simulink library "Load_Lib"  (R2025a)
settings: Solver=ode45  StartTime=0.0  StopTime=10.0  RelTol=1e-3  EnableMultiTasking=on
undefined symbols (not defined in the file or in its folder): Local, Scissor_Lift_Param, X, Y, Z
libraries: sm_lib x41, Scissor_Parts_Lib x24, fl_lib x6
(part 1 of 2)
Description:
  | Copyright 2015-2025 The MathWorks, Inc.
settings Model: Creator=smiller  LastModifiedBy=smiller
settings SolverCC: AlgebraicLoopSolver=TrustRegion
settings DataIOCC: LimitDataPoints=on  SaveFormat=Array  ReturnWorkspaceOutputs=off
settings OptimizationCC: ReuseModelBlockBuffer=off  ExpressionDepthLimit=2147483647.0  LifeSpan=inf
settings DebuggingCC: UnderspecifiedInitializationDetection=Classic  MergeDetectMultiDrivingBlocksExec=none  SolverPrmCheckMsg=warning  UnconnectedInputMsg=warning  UnconnectedOutputMsg=warning  UnconnectedLineMsg=warning  AllowSymbolicDim=off  StateNameClashWarn=warning  PregeneratedLibrarySubsystemCodeDiagnostic=none  SFUnexpectedBacktrackingDiag=warning  SFNoUnconditionalDefaultTransitionDiag=warning  SFExecutionAtInitializationDiag=none  ArithmeticOperatorsInVariantConditions=warning
settings HardwareCC: ProdBitPerPointer=32.0  ProdBitPerSizeT=32.0  ProdBitPerPtrDiffT=32.0  ProdLargestAtomicFloat=None  ProdIntDivRoundTo=Undefined  ProdEndianess=Unspecified  ProdWordSize=32.0  ProdHWDeviceType=32-bit Generic
settings ModelReferenceCC: EnableRefExpFcnMdlSchedulingChecks=on  PropagateSignalLabelsOutOfModel=off
settings SFSimCC: SimUseLocalCustomCode=off  CustomCodeUndefinedFunction=UseInterfaceOnly
settings RTWCC: RTWUseLocalCustomCode=off  GPUComputeCapability=3.5  DLArmComputeVersion=19.05
settings CodeAppCC: StateflowObjectComments=on
settings GRTTargetCC: TargetLangStandard=C89/C90 (ANSI)
settings ConfigComp: CovMetricSettings=dw  CovSaveCumulativeToWorkspaceVar=on  CovSaveSingleToWorkspaceVar=on  CovExternalEMLEnable=off  CovSFcnEnable=off

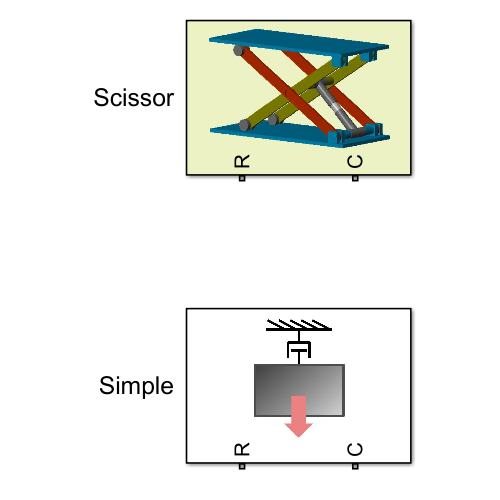
[thumbnail: Simulink's stored preview of the top-level diagram]
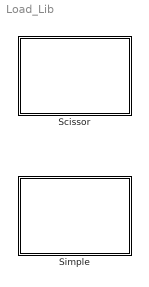
== system Load_Lib ==
  Scissor : Subsystem
      mask Display: image('Load_Scissor_IMAGE.JPG');
  Simple : Subsystem
      mask Display: image('Load_Simple_IMAGE.JPG');

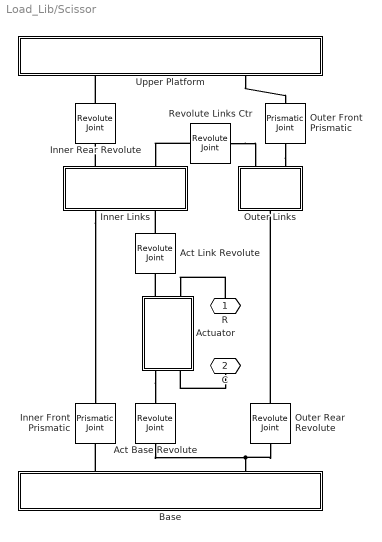
== system Load_Lib/Scissor ==
  Act Base Revolute : sm_lib/Joints/Revolute Joint  JointMode=Normal  CompositeWrenchDir=FollowerOnBase  CompositeWrenchFrame=BaseFrame  SenseConstraintForce=off  SenseConstraintTorque=off  SenseTotalForce=off  SenseTotalTorque=off  PositionTargetSpecify=off  PositionTargetPriority=High  PositionTargetValue=0  PositionTargetValueUnits=deg  VelocityTargetSpecify=off  VelocityTargetPriority=High  VelocityTargetValue=0  VelocityTargetValueUnits=deg/s  EquilibriumPosition=0  EquilibriumPositionUnits=deg  SpringStiffness=0  SpringStiffnessUnits=N*m/deg  DampingCoefficient=0  DampingCoefficientUnits=N*m/(deg/s)  LowerLimitSpecify=off  LowerLimitBound=-90  LowerLimitBoundUnits=deg  LowerLimitStiffness=1e4  LowerLimitStiffnessUnits=N*m/deg  LowerLimitDamping=10  LowerLimitDampingUnits=N*m/(deg/s)  LowerLimitTransitionRegionWidth=0.1  LowerLimitTransitionRegionWidthUnits=deg  UpperLimitSpecify=off  UpperLimitBound=90  UpperLimitBoundUnits=deg  UpperLimitStiffness=1e4  UpperLimitStiffnessUnits=N*m/deg  UpperLimitDamping=10  UpperLimitDampingUnits=N*m/(deg/s)  UpperLimitTransitionRegionWidth=0.1  UpperLimitTransitionRegionWidthUnits=deg  TorqueActuationMode=NoTorque  MotionActuationMode=ComputedMotion  SensePosition=off  SenseVelocity=off  SenseAcceleration=off  SenseTorqueForce=off  SenseLowerLimitTorqueForce=off  SenseUpperLimitTorqueForce=off
  Act Link Revolute : sm_lib/Joints/Revolute Joint  JointMode=Normal  CompositeWrenchDir=FollowerOnBase  CompositeWrenchFrame=BaseFrame  SenseConstraintForce=off  SenseConstraintTorque=off  SenseTotalForce=off  SenseTotalTorque=off  PositionTargetSpecify=off  PositionTargetPriority=High  PositionTargetValue=0  PositionTargetValueUnits=deg  VelocityTargetSpecify=off  VelocityTargetPriority=High  VelocityTargetValue=0  VelocityTargetValueUnits=deg/s  EquilibriumPosition=0  EquilibriumPositionUnits=deg  SpringStiffness=0  SpringStiffnessUnits=N*m/deg  DampingCoefficient=0  DampingCoefficientUnits=N*m/(deg/s)  LowerLimitSpecify=off  LowerLimitBound=-90  LowerLimitBoundUnits=deg  LowerLimitStiffness=1e4  LowerLimitStiffnessUnits=N*m/deg  LowerLimitDamping=10  LowerLimitDampingUnits=N*m/(deg/s)  LowerLimitTransitionRegionWidth=0.1  LowerLimitTransitionRegionWidthUnits=deg  UpperLimitSpecify=off  UpperLimitBound=90  UpperLimitBoundUnits=deg  UpperLimitStiffness=1e4  UpperLimitStiffnessUnits=N*m/deg  UpperLimitDamping=10  UpperLimitDampingUnits=N*m/(deg/s)  UpperLimitTransitionRegionWidth=0.1  UpperLimitTransitionRegionWidthUnits=deg  TorqueActuationMode=NoTorque  MotionActuationMode=ComputedMotion  SensePosition=off  SenseVelocity=off  SenseAcceleration=off  SenseTorqueForce=off  SenseLowerLimitTorqueForce=off  SenseUpperLimitTorqueForce=off
  Actuator : Subsystem
  Base : Subsystem
  Inner Links : Subsystem
  "Inner Front Prismatic " : sm_lib/Joints/Prismatic Joint  JointMode=Normal  CompositeWrenchDir=FollowerOnBase  CompositeWrenchFrame=BaseFrame  SenseConstraintForce=off  SenseConstraintTorque=off  SenseTotalForce=off  SenseTotalTorque=off  PositionTargetSpecify=off  PositionTargetPriority=High  PositionTargetValue=0  PositionTargetValueUnits=m  VelocityTargetSpecify=off  VelocityTargetPriority=High  VelocityTargetValue=0  VelocityTargetValueUnits=m/s  EquilibriumPosition=0  EquilibriumPositionUnits=m  SpringStiffness=0  SpringStiffnessUnits=N/m  DampingCoefficient=0  DampingCoefficientUnits=N/(m/s)  LowerLimitSpecify=off  LowerLimitBound=-1  LowerLimitBoundUnits=m  LowerLimitStiffness=1e6  LowerLimitStiffnessUnits=N/m  LowerLimitDamping=1e3  LowerLimitDampingUnits=N/(m/s)  LowerLimitTransitionRegionWidth=1e-4  LowerLimitTransitionRegionWidthUnits=m  UpperLimitSpecify=off  UpperLimitBound=1  UpperLimitBoundUnits=m  UpperLimitStiffness=1e6  UpperLimitStiffnessUnits=N/m  UpperLimitDamping=1e3  UpperLimitDampingUnits=N/(m/s)  UpperLimitTransitionRegionWidth=1e-4  UpperLimitTransitionRegionWidthUnits=m  TorqueActuationMode=NoTorque  MotionActuationMode=ComputedMotion  SensePosition=off  SenseVelocity=off  SenseAcceleration=off  SenseTorqueForce=off  SenseLowerLimitTorqueForce=off  SenseUpperLimitTorqueForce=off
  Inner Rear Revolute : sm_lib/Joints/Revolute Joint  JointMode=Normal  CompositeWrenchDir=FollowerOnBase  CompositeWrenchFrame=BaseFrame  SenseConstraintForce=off  SenseConstraintTorque=off  SenseTotalForce=off  SenseTotalTorque=off  PositionTargetSpecify=off  PositionTargetPriority=Low  PositionTargetValue=15  PositionTargetValueUnits=deg  VelocityTargetSpecify=off  VelocityTargetPriority=High  VelocityTargetValue=0  VelocityTargetValueUnits=deg/s  EquilibriumPosition=0  EquilibriumPositionUnits=deg  SpringStiffness=0  SpringStiffnessUnits=N*m/deg  DampingCoefficient=0  DampingCoefficientUnits=N*m/(deg/s)  LowerLimitSpecify=off  LowerLimitBound=-90  LowerLimitBoundUnits=deg  LowerLimitStiffness=1e4  LowerLimitStiffnessUnits=N*m/deg  LowerLimitDamping=10  LowerLimitDampingUnits=N*m/(deg/s)  LowerLimitTransitionRegionWidth=0.1  LowerLimitTransitionRegionWidthUnits=deg  UpperLimitSpecify=off  UpperLimitBound=90  UpperLimitBoundUnits=deg  UpperLimitStiffness=1e4  UpperLimitStiffnessUnits=N*m/deg  UpperLimitDamping=10  UpperLimitDampingUnits=N*m/(deg/s)  UpperLimitTransitionRegionWidth=0.1  UpperLimitTransitionRegionWidthUnits=deg  TorqueActuationMode=NoTorque  MotionActuationMode=ComputedMotion  SensePosition=off  SenseVelocity=off  SenseAcceleration=off  SenseTorqueForce=off  SenseLowerLimitTorqueForce=off  SenseUpperLimitTorqueForce=off
  Outer Links : Subsystem
  "Outer Front Prismatic " : sm_lib/Joints/Prismatic Joint  JointMode=Normal  CompositeWrenchDir=FollowerOnBase  CompositeWrenchFrame=BaseFrame  SenseConstraintForce=off  SenseConstraintTorque=off  SenseTotalForce=off  SenseTotalTorque=off  PositionTargetSpecify=off  PositionTargetPriority=High  PositionTargetValue=0  PositionTargetValueUnits=m  VelocityTargetSpecify=off  VelocityTargetPriority=High  VelocityTargetValue=0  VelocityTargetValueUnits=m/s  EquilibriumPosition=0  EquilibriumPositionUnits=m  SpringStiffness=0  SpringStiffnessUnits=N/m  DampingCoefficient=0  DampingCoefficientUnits=N/(m/s)  LowerLimitSpecify=off  LowerLimitBound=-1  LowerLimitBoundUnits=m  LowerLimitStiffness=1e6  LowerLimitStiffnessUnits=N/m  LowerLimitDamping=1e3  LowerLimitDampingUnits=N/(m/s)  LowerLimitTransitionRegionWidth=1e-4  LowerLimitTransitionRegionWidthUnits=m  UpperLimitSpecify=off  UpperLimitBound=1  UpperLimitBoundUnits=m  UpperLimitStiffness=1e6  UpperLimitStiffnessUnits=N/m  UpperLimitDamping=1e3  UpperLimitDampingUnits=N/(m/s)  UpperLimitTransitionRegionWidth=1e-4  UpperLimitTransitionRegionWidthUnits=m  TorqueActuationMode=NoTorque  MotionActuationMode=ComputedMotion  SensePosition=off  SenseVelocity=off  SenseAcceleration=off  SenseTorqueForce=off  SenseLowerLimitTorqueForce=off  SenseUpperLimitTorqueForce=off
  Outer Rear Revolute : sm_lib/Joints/Revolute Joint  JointMode=Normal  CompositeWrenchDir=FollowerOnBase  CompositeWrenchFrame=BaseFrame  SenseConstraintForce=off  SenseConstraintTorque=off  SenseTotalForce=off  SenseTotalTorque=off  PositionTargetSpecify=off  PositionTargetPriority=Low  PositionTargetValue=-15  PositionTargetValueUnits=deg  VelocityTargetSpecify=off  VelocityTargetPriority=High  VelocityTargetValue=0  VelocityTargetValueUnits=deg/s  EquilibriumPosition=0  EquilibriumPositionUnits=deg  SpringStiffness=0  SpringStiffnessUnits=N*m/deg  DampingCoefficient=0  DampingCoefficientUnits=N*m/(deg/s)  LowerLimitSpecify=off  LowerLimitBound=-90  LowerLimitBoundUnits=deg  LowerLimitStiffness=1e4  LowerLimitStiffnessUnits=N*m/deg  LowerLimitDamping=10  LowerLimitDampingUnits=N*m/(deg/s)  LowerLimitTransitionRegionWidth=0.1  LowerLimitTransitionRegionWidthUnits=deg  UpperLimitSpecify=off  UpperLimitBound=90  UpperLimitBoundUnits=deg  UpperLimitStiffness=1e4  UpperLimitStiffnessUnits=N*m/deg  UpperLimitDamping=10  UpperLimitDampingUnits=N*m/(deg/s)  UpperLimitTransitionRegionWidth=0.1  UpperLimitTransitionRegionWidthUnits=deg  TorqueActuationMode=NoTorque  MotionActuationMode=ComputedMotion  SensePosition=off  SenseVelocity=off  SenseAcceleration=off  SenseTorqueForce=off  SenseLowerLimitTorqueForce=off  SenseUpperLimitTorqueForce=off
  Revolute Links Ctr : sm_lib/Joints/Revolute Joint  JointMode=Normal  CompositeWrenchDir=FollowerOnBase  CompositeWrenchFrame=BaseFrame  SenseConstraintForce=off  SenseConstraintTorque=off  SenseTotalForce=off  SenseTotalTorque=off  PositionTargetSpecify=on  PositionTargetPriority=Low  PositionTargetValue=-2*Scissor_Lift_Param.Initial_Angle  PositionTargetValueUnits=deg  VelocityTargetSpecify=off  VelocityTargetPriority=High  VelocityTargetValue=0  VelocityTargetValueUnits=deg/s  EquilibriumPosition=0  EquilibriumPositionUnits=deg  SpringStiffness=0  SpringStiffnessUnits=N*m/deg  DampingCoefficient=0  DampingCoefficientUnits=N*m/(deg/s)  LowerLimitSpecify=off  LowerLimitBound=-90  LowerLimitBoundUnits=deg  LowerLimitStiffness=1e4  LowerLimitStiffnessUnits=N*m/deg  LowerLimitDamping=10  LowerLimitDampingUnits=N*m/(deg/s)  LowerLimitTransitionRegionWidth=0.1  LowerLimitTransitionRegionWidthUnits=deg  UpperLimitSpecify=off  UpperLimitBound=90  UpperLimitBoundUnits=deg  UpperLimitStiffness=1e4  UpperLimitStiffnessUnits=N*m/deg  UpperLimitDamping=10  UpperLimitDampingUnits=N*m/(deg/s)  UpperLimitTransitionRegionWidth=0.1  UpperLimitTransitionRegionWidthUnits=deg  TorqueActuationMode=NoTorque  MotionActuationMode=ComputedMotion  SensePosition=off  SenseVelocity=off  SenseAcceleration=off  SenseTorqueForce=off  SenseLowerLimitTorqueForce=off  SenseUpperLimitTorqueForce=off
  Upper Platform : Subsystem
  R : PMIOPort  Side=Left
  C : PMIOPort  Port=2  Side=Left
  connections:
  R/RConn1 -- Actuator/RConn2
  C/RConn1 -- Actuator/LConn2
  Actuator/LConn1 -- Act Base Revolute/RConn1
  Act Link Revolute/LConn1 -- Inner Links/RConn2
  Actuator/RConn1 -- Act Link Revolute/RConn1
  Revolute Links Ctr/LConn1 -- Inner Links/LConn2
  Revolute Links Ctr/RConn1 -- Outer Links/RConn1
  Outer Rear Revolute/RConn1 -- Outer Links/LConn1
  Inner Links/LConn1 -- Inner Rear Revolute/RConn1
  Inner Rear Revolute/LConn1 -- Upper Platform/LConn1
  "Outer Front Prismatic "/LConn1 -- Outer Links/RConn2
  Upper Platform/LConn2 -- "Outer Front Prismatic "/RConn1
  Base/RConn1 -- "Inner Front Prismatic "/RConn1
  Inner Links/RConn1 -- "Inner Front Prismatic "/LConn1
  Outer Rear Revolute/LConn1 -- Base/RConn2 -- Act Base Revolute/LConn1

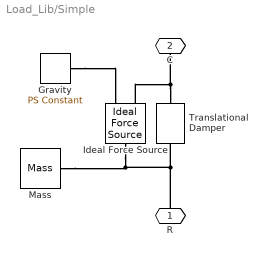
== system Load_Lib/Simple ==
  Gravity : fl_lib/Physical Signals/Sources/PS Constant  constant=9.81*Scissor_Lift_Param.Load.Mass N
  Ideal Force Source : fl_lib/Mechanical/Mechanical Sources/Ideal Force Source
  Mass : fl_lib/Mechanical/Translational Elements/Mass  mass=Scissor_Lift_Param.Load.Mass kg  num_ports=foundation.enum.numPorts2.one  v_specify=on  v_priority=High  v=0 m/s  v_nominal_specify=off  v_nominal_value=1  v_nominal_unit=m/s  f_specify=off  f_priority=High  f=0 N  f_nominal_specify=off  f_nominal_value=1  f_nominal_unit=N
  Translational Damper : fl_lib/Mechanical/Translational Elements/Translational Damper  D=Scissor_Lift_Param.Actuator.Damping N/(m/s)  v_specify=off  v_priority=High  v=0 m/s  v_nominal_specify=off  v_nominal_value=1  v_nominal_unit=m/s  f_specify=off  f_priority=High  f=0 N  f_nominal_specify=off  f_nominal_value=1  f_nominal_unit=N
  R : PMIOPort  Side=Left
  C : PMIOPort  Port=2  Side=Left
  connections:
  Translational Damper/LConn1 -- R/RConn1 -- Ideal Force Source/LConn1 -- Mass/LConn1
  Translational Damper/RConn1 -- C/RConn1 -- Ideal Force Source/RConn2
  Gravity/RConn1 -- Ideal Force Source/RConn1

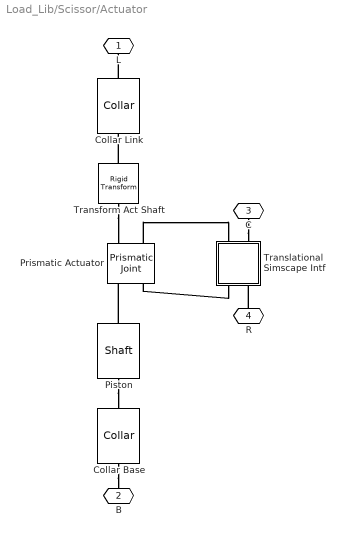
== system Load_Lib/Scissor/Actuator ==
  Collar Base : Scissor_Parts_Lib/Collar  collar_length=Scissor_Lift_Param.Actuator.Collar.Length  collar_radius=Scissor_Lift_Param.Actuator.Collar.Radius  cylinder_length=Scissor_Lift_Param.Actuator.Piston_Seat.Length*2  cylinder_radius=Scissor_Lift_Param.Actuator.Piston_Seat.Radius  cylinder_ori=Local +Z  material_density=Scissor_Lift_Param.Actuator.Collar.Density  material_color=Scissor_Lift_Param.Actuator.Collar.Color  material_opacity=Scissor_Lift_Param.Actuator.Collar.Opacity
  Collar Link : Scissor_Parts_Lib/Collar  collar_length=Scissor_Lift_Param.Actuator.Collar.Length  collar_radius=Scissor_Lift_Param.Actuator.Collar.Radius  cylinder_length=Scissor_Lift_Param.Actuator.Piston_Seat.Length*2  cylinder_radius=Scissor_Lift_Param.Actuator.Piston_Seat.Radius  cylinder_ori=Local +Z  material_density=Scissor_Lift_Param.Actuator.Collar.Density  material_color=Scissor_Lift_Param.Actuator.Collar.Color  material_opacity=Scissor_Lift_Param.Actuator.Collar.Opacity
  Piston : Scissor_Parts_Lib/Shaft  L=Scissor_Lift_Param.Actuator.Piston.Length  r=Scissor_Lift_Param.Actuator.Piston.Radius  theta=0  z_ori=Local +Z  Ro=Scissor_Lift_Param.Actuator.Piston.Density  clr=Scissor_Lift_Param.Actuator.Piston.Color  opc=Scissor_Lift_Param.Actuator.Piston.Opacity
  Prismatic Actuator : sm_lib/Joints/Prismatic Joint  JointMode=Normal  CompositeWrenchDir=FollowerOnBase  CompositeWrenchFrame=BaseFrame  SenseConstraintForce=off  SenseConstraintTorque=off  SenseTotalForce=off  SenseTotalTorque=off  PositionTargetSpecify=off  PositionTargetPriority=High  PositionTargetValue=0  PositionTargetValueUnits=m  VelocityTargetSpecify=off  VelocityTargetPriority=High  VelocityTargetValue=0  VelocityTargetValueUnits=m/s  EquilibriumPosition=0  EquilibriumPositionUnits=m  SpringStiffness=0  SpringStiffnessUnits=N/m  DampingCoefficient=Scissor_Lift_Param.Actuator.Damping  DampingCoefficientUnits=N/(m/s)  LowerLimitSpecify=off  LowerLimitBound=-1  LowerLimitBoundUnits=m  LowerLimitStiffness=1e6  LowerLimitStiffnessUnits=N/m  LowerLimitDamping=1e3  LowerLimitDampingUnits=N/(m/s)  LowerLimitTransitionRegionWidth=1e-4  LowerLimitTransitionRegionWidthUnits=m  UpperLimitSpecify=off  UpperLimitBound=1  UpperLimitBoundUnits=m  UpperLimitStiffness=1e6  UpperLimitStiffnessUnits=N/m  UpperLimitDamping=1e3  UpperLimitDampingUnits=N/(m/s)  UpperLimitTransitionRegionWidth=1e-4  UpperLimitTransitionRegionWidthUnits=m  TorqueActuationMode=InputTorque  MotionActuationMode=ComputedMotion  SensePosition=off  SenseVelocity=on  SenseAcceleration=off  SenseTorqueForce=off  SenseLowerLimitTorqueForce=off  SenseUpperLimitTorqueForce=off
  Transform Act Shaft : sm_lib/Frames and Transforms/Rigid Transform  RotationMethod=StandardAxis  FollAlignAxisA=+X  BaseAlignAxisA=+Y  FollAlignAxisB=+Y  BaseAlignAxisB=+Z  RotationStandardAxis=+X  RotationAngle=180  RotationAngleUnits=deg  RotationArbitraryAxis=[0 0 1]  RotationSequenceAxes=FollowerAxes  RotationSequence=XYX  RotationSequenceAngles=[0 0 0]  RotationSequenceAnglesUnits=deg  RotationMatrix=[1 0 0; 0 1 0; 0 0 1]  Quaternion=[1 0 0 0]  TranslationMethod=None  TranslationCartesianOffset=[0 0 0]  TranslationCartesianOffsetUnits=cm  TranslationStandardAxis=-X  TranslationStandardOffset=0  TranslationStandardOffsetUnits=cm  TranslationROffset=0  TranslationROffsetUnits=m  TranslationThetaOffset=0  TranslationThetaOffsetUnits=deg  TranslationZOffset=0  TranslationZOffsetUnits=m
  Translational Simscape Intf : Subsystem
  L : PMIOPort  Side=Right
  B : PMIOPort  Port=2  Side=Left
  C : PMIOPort  Port=3  Side=Left
  R : PMIOPort  Port=4  Side=Right
  connections:
  R/RConn1 -- Translational Simscape Intf/RConn2
  C/RConn1 -- Translational Simscape Intf/LConn2
  Piston/RConn1 -- Prismatic Actuator/RConn1
  Piston/LConn1 -- Collar Base/RConn1
  Transform Act Shaft/LConn1 -- Collar Link/RConn1
  Collar Link/LConn1 -- L/RConn1
  Translational Simscape Intf/RConn1 -- Prismatic Actuator/RConn2
  Prismatic Actuator/LConn2 -- Translational Simscape Intf/LConn1
  Transform Act Shaft/RConn1 -- Prismatic Actuator/LConn1
  Collar Base/LConn1 -- B/RConn1

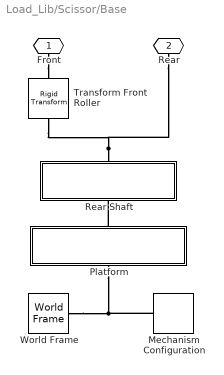
== system Load_Lib/Scissor/Base ==
  Mechanism Configuration : sm_lib/Utilities/Mechanism Configuration  UniformGravity=Constant  GravityVector=[0 0 -9.81]  GravityVectorUnits=m/s^2  LinearizationDelta=0.001  JointModeTransitionNonlinearIterations=2
  Platform : Subsystem
  Rear Shaft : Subsystem
  Transform Front Roller : sm_lib/Frames and Transforms/Rigid Transform  RotationMethod=StandardAxis  FollAlignAxisA=+X  BaseAlignAxisA=+Y  FollAlignAxisB=+Y  BaseAlignAxisB=+Z  RotationStandardAxis=+Y  RotationAngle=90  RotationAngleUnits=deg  RotationArbitraryAxis=[0 0 1]  RotationSequenceAxes=FollowerAxes  RotationSequence=XYX  RotationSequenceAngles=[0 0 0]  RotationSequenceAnglesUnits=deg  RotationMatrix=[1 0 0; 0 1 0; 0 0 1]  Quaternion=[1 0 0 0]  TranslationMethod=Cartesian  TranslationCartesianOffset=[-Scissor_Lift_Param.Link.Length -Scissor_Lift_Param.Base_Block.Height/2 0]  TranslationCartesianOffsetUnits=cm  TranslationStandardAxis=-X  TranslationStandardOffset=0  TranslationStandardOffsetUnits=cm  TranslationROffset=0  TranslationROffsetUnits=m  TranslationThetaOffset=0  TranslationThetaOffsetUnits=deg  TranslationZOffset=0  TranslationZOffsetUnits=m
  World Frame : sm_lib/Frames and Transforms/World Frame
  Front : PMIOPort  Side=Right
  Rear : PMIOPort  Port=2  Side=Right
  connections:
  Platform/RConn1 -- Rear Shaft/LConn1
  Platform/LConn1 -- Mechanism Configuration/RConn1 -- World Frame/RConn1
  Rear Shaft/RConn1 -- Transform Front Roller/LConn1 -- Rear/RConn1
  Front/RConn1 -- Transform Front Roller/RConn1

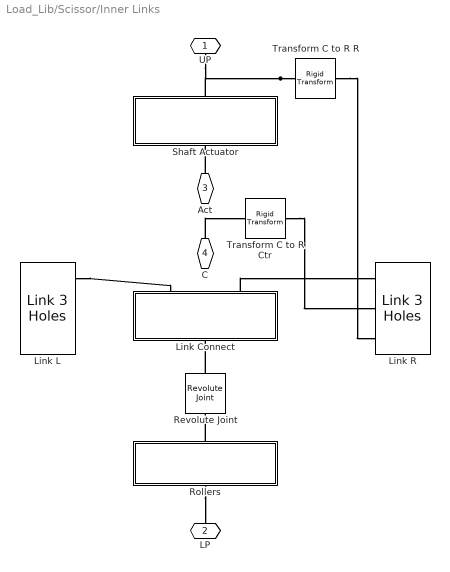
== system Load_Lib/Scissor/Inner Links ==
  Link Connect : Subsystem
  Link L : Scissor_Parts_Lib/Link 3 Holes  L=Scissor_Lift_Param.Link.Length  W=Scissor_Lift_Param.Link.Width  T=Scissor_Lift_Param.Link.Thickness  r=Scissor_Lift_Param.Link.Hole_Radius  rho=Scissor_Lift_Param.Link.Density  clr_string=Yellow  opc=Scissor_Lift_Param.Link.Opacity
  Link R : Scissor_Parts_Lib/Link 3 Holes  L=Scissor_Lift_Param.Link.Length  W=Scissor_Lift_Param.Link.Width  T=Scissor_Lift_Param.Link.Thickness  r=Scissor_Lift_Param.Link.Hole_Radius  rho=Scissor_Lift_Param.Link.Density  clr_string=Yellow  opc=Scissor_Lift_Param.Link.Opacity
  Revolute Joint : sm_lib/Joints/Revolute Joint  JointMode=Normal  CompositeWrenchDir=FollowerOnBase  CompositeWrenchFrame=BaseFrame  SenseConstraintForce=off  SenseConstraintTorque=off  SenseTotalForce=off  SenseTotalTorque=off  PositionTargetSpecify=off  PositionTargetPriority=High  PositionTargetValue=0  PositionTargetValueUnits=deg  VelocityTargetSpecify=off  VelocityTargetPriority=High  VelocityTargetValue=0  VelocityTargetValueUnits=deg/s  EquilibriumPosition=0  EquilibriumPositionUnits=deg  SpringStiffness=0  SpringStiffnessUnits=N*m/deg  DampingCoefficient=0  DampingCoefficientUnits=N*m/(deg/s)  LowerLimitSpecify=off  LowerLimitBound=-90  LowerLimitBoundUnits=deg  LowerLimitStiffness=1e4  LowerLimitStiffnessUnits=N*m/deg  LowerLimitDamping=10  LowerLimitDampingUnits=N*m/(deg/s)  LowerLimitTransitionRegionWidth=0.1  LowerLimitTransitionRegionWidthUnits=deg  UpperLimitSpecify=off  UpperLimitBound=90  UpperLimitBoundUnits=deg  UpperLimitStiffness=1e4  UpperLimitStiffnessUnits=N*m/deg  UpperLimitDamping=10  UpperLimitDampingUnits=N*m/(deg/s)  UpperLimitTransitionRegionWidth=0.1  UpperLimitTransitionRegionWidthUnits=deg  TorqueActuationMode=NoTorque  MotionActuationMode=ComputedMotion  SensePosition=off  SenseVelocity=off  SenseAcceleration=off  SenseTorqueForce=off  SenseLowerLimitTorqueForce=off  SenseUpperLimitTorqueForce=off
  Rollers : Subsystem
  Shaft Actuator : Subsystem
  Transform C to R Ctr : sm_lib/Frames and Transforms/Rigid Transform  RotationMethod=None  FollAlignAxisA=+X  BaseAlignAxisA=+Y  FollAlignAxisB=+Y  BaseAlignAxisB=+Z  RotationStandardAxis=+X  RotationAngle=90  RotationAngleUnits=deg  RotationArbitraryAxis=[0 0 1]  RotationSequenceAxes=FollowerAxes  RotationSequence=XYX  RotationSequenceAngles=[0 0 0]  RotationSequenceAnglesUnits=deg  RotationMatrix=[1 0 0; 0 1 0; 0 0 1]  Quaternion=[1 0 0 0]  TranslationMethod=StandardAxis  TranslationCartesianOffset=[0 0 0]  TranslationCartesianOffsetUnits=cm  TranslationStandardAxis=-Z  TranslationStandardOffset=Scissor_Lift_Param.Link_Separation.Inner_Inner/2  TranslationStandardOffsetUnits=cm  TranslationROffset=0  TranslationROffsetUnits=m  TranslationThetaOffset=0  TranslationThetaOffsetUnits=deg  TranslationZOffset=0  TranslationZOffsetUnits=m
  Transform C to R R : sm_lib/Frames and Transforms/Rigid Transform  RotationMethod=None  FollAlignAxisA=+X  BaseAlignAxisA=+Y  FollAlignAxisB=+Y  BaseAlignAxisB=+Z  RotationStandardAxis=+X  RotationAngle=90  RotationAngleUnits=deg  RotationArbitraryAxis=[0 0 1]  RotationSequenceAxes=FollowerAxes  RotationSequence=XYX  RotationSequenceAngles=[0 0 0]  RotationSequenceAnglesUnits=deg  RotationMatrix=[1 0 0; 0 1 0; 0 0 1]  Quaternion=[1 0 0 0]  TranslationMethod=StandardAxis  TranslationCartesianOffset=[0 0 0]  TranslationCartesianOffsetUnits=cm  TranslationStandardAxis=-Z  TranslationStandardOffset=Scissor_Lift_Param.Link_Separation.Inner_Inner/2  TranslationStandardOffsetUnits=cm  TranslationROffset=0  TranslationROffsetUnits=m  TranslationThetaOffset=0  TranslationThetaOffsetUnits=deg  TranslationZOffset=0  TranslationZOffsetUnits=m
  UP : PMIOPort  Side=Left
  LP : PMIOPort  Port=2  Side=Right
  Act : PMIOPort  Port=3  Side=Right
  C : PMIOPort  Port=4  Side=Left
  connections:
  Revolute Joint/LConn1 -- Link Connect/LConn1
  Link L/RConn1 -- Link Connect/RConn1
  Link Connect/RConn2 -- Link R/RConn1
  Act/RConn1 -- Shaft Actuator/RConn1
  Rollers/LConn1 -- LP/RConn1
  Rollers/RConn1 -- Revolute Joint/RConn1
  C/RConn1 -- Transform C to R Ctr/LConn1
  Transform C to R Ctr/RConn1 -- Link R/RConn2
  Transform C to R R/LConn1 -- Shaft Actuator/LConn1 -- UP/RConn1
  Transform C to R R/RConn1 -- Link R/RConn3

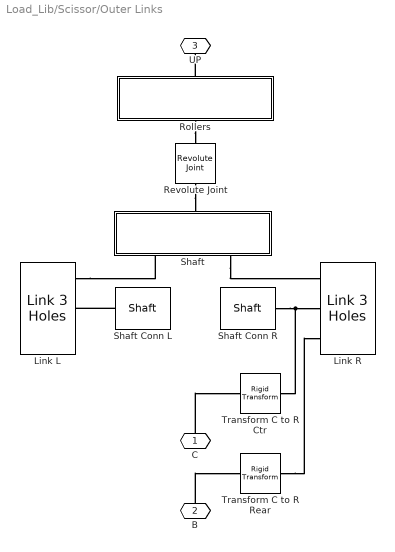
== system Load_Lib/Scissor/Outer Links ==
  Link L : Scissor_Parts_Lib/Link 3 Holes  L=Scissor_Lift_Param.Link.Length  W=Scissor_Lift_Param.Link.Width  T=Scissor_Lift_Param.Link.Thickness  r=Scissor_Lift_Param.Link.Hole_Radius  rho=Scissor_Lift_Param.Link.Density  clr_string=Red  opc=Scissor_Lift_Param.Link.Opacity
  Link R : Scissor_Parts_Lib/Link 3 Holes  L=Scissor_Lift_Param.Link.Length  W=Scissor_Lift_Param.Link.Width  T=Scissor_Lift_Param.Link.Thickness  r=Scissor_Lift_Param.Link.Hole_Radius  rho=Scissor_Lift_Param.Link.Density  clr_string=Red  opc=Scissor_Lift_Param.Link.Opacity
  Revolute Joint : sm_lib/Joints/Revolute Joint  JointMode=Normal  CompositeWrenchDir=FollowerOnBase  CompositeWrenchFrame=BaseFrame  SenseConstraintForce=off  SenseConstraintTorque=off  SenseTotalForce=off  SenseTotalTorque=off  PositionTargetSpecify=off  PositionTargetPriority=High  PositionTargetValue=0  PositionTargetValueUnits=deg  VelocityTargetSpecify=off  VelocityTargetPriority=High  VelocityTargetValue=0  VelocityTargetValueUnits=deg/s  EquilibriumPosition=0  EquilibriumPositionUnits=deg  SpringStiffness=0  SpringStiffnessUnits=N*m/deg  DampingCoefficient=0  DampingCoefficientUnits=N*m/(deg/s)  LowerLimitSpecify=off  LowerLimitBound=-90  LowerLimitBoundUnits=deg  LowerLimitStiffness=1e4  LowerLimitStiffnessUnits=N*m/deg  LowerLimitDamping=10  LowerLimitDampingUnits=N*m/(deg/s)  LowerLimitTransitionRegionWidth=0.1  LowerLimitTransitionRegionWidthUnits=deg  UpperLimitSpecify=off  UpperLimitBound=90  UpperLimitBoundUnits=deg  UpperLimitStiffness=1e4  UpperLimitStiffnessUnits=N*m/deg  UpperLimitDamping=10  UpperLimitDampingUnits=N*m/(deg/s)  UpperLimitTransitionRegionWidth=0.1  UpperLimitTransitionRegionWidthUnits=deg  TorqueActuationMode=NoTorque  MotionActuationMode=ComputedMotion  SensePosition=off  SenseVelocity=off  SenseAcceleration=off  SenseTorqueForce=off  SenseLowerLimitTorqueForce=off  SenseUpperLimitTorqueForce=off
  Rollers : Subsystem
  Shaft : Subsystem
  Shaft Conn L : Scissor_Parts_Lib/Shaft  L=Scissor_Lift_Param.Conn_Shaft.Length  r=Scissor_Lift_Param.Trans_Shaft.Radius  theta=0  z_ori=Local -Z  Ro=Scissor_Lift_Param.Trans_Shaft.Density  clr=Scissor_Lift_Param.Conn_Shaft.Color  opc=Scissor_Lift_Param.Trans_Shaft.Opacity
  Shaft Conn R : Scissor_Parts_Lib/Shaft  L=Scissor_Lift_Param.Conn_Shaft.Length  r=Scissor_Lift_Param.Trans_Shaft.Radius  theta=0  z_ori=Local +Z  Ro=Scissor_Lift_Param.Trans_Shaft.Density  clr=Scissor_Lift_Param.Conn_Shaft.Color  opc=Scissor_Lift_Param.Trans_Shaft.Opacity
  Transform C to R Ctr : sm_lib/Frames and Transforms/Rigid Transform  RotationMethod=None  FollAlignAxisA=+X  BaseAlignAxisA=+Y  FollAlignAxisB=+Y  BaseAlignAxisB=+Z  RotationStandardAxis=+X  RotationAngle=90  RotationAngleUnits=deg  RotationArbitraryAxis=[0 0 1]  RotationSequenceAxes=FollowerAxes  RotationSequence=XYX  RotationSequenceAngles=[0 0 0]  RotationSequenceAnglesUnits=deg  RotationMatrix=[1 0 0; 0 1 0; 0 0 1]  Quaternion=[1 0 0 0]  TranslationMethod=StandardAxis  TranslationCartesianOffset=[0 0 0]  TranslationCartesianOffsetUnits=cm  TranslationStandardAxis=-Z  TranslationStandardOffset=Scissor_Lift_Param.Link_Separation.Outer_Outer/2  TranslationStandardOffsetUnits=cm  TranslationROffset=0  TranslationROffsetUnits=m  TranslationThetaOffset=0  TranslationThetaOffsetUnits=deg  TranslationZOffset=0  TranslationZOffsetUnits=m
  "Transform C to R Rear " : sm_lib/Frames and Transforms/Rigid Transform  RotationMethod=None  FollAlignAxisA=+X  BaseAlignAxisA=+Y  FollAlignAxisB=+Y  BaseAlignAxisB=+Z  RotationStandardAxis=+X  RotationAngle=90  RotationAngleUnits=deg  RotationArbitraryAxis=[0 0 1]  RotationSequenceAxes=FollowerAxes  RotationSequence=XYX  RotationSequenceAngles=[0 0 0]  RotationSequenceAnglesUnits=deg  RotationMatrix=[1 0 0; 0 1 0; 0 0 1]  Quaternion=[1 0 0 0]  TranslationMethod=StandardAxis  TranslationCartesianOffset=[0 0 0]  TranslationCartesianOffsetUnits=cm  TranslationStandardAxis=-Z  TranslationStandardOffset=Scissor_Lift_Param.Link_Separation.Outer_Outer/2  TranslationStandardOffsetUnits=cm  TranslationROffset=0  TranslationROffsetUnits=m  TranslationThetaOffset=0  TranslationThetaOffsetUnits=deg  TranslationZOffset=0  TranslationZOffsetUnits=m
  C : PMIOPort  Side=Right
  B : PMIOPort  Port=2  Side=Left
  UP : PMIOPort  Port=3  Side=Right
  connections:
  Shaft Conn L/LConn1 -- Link L/RConn2
  Shaft/RConn2 -- Link R/RConn1
  Link L/RConn1 -- Shaft/RConn1
  Revolute Joint/LConn1 -- Shaft/LConn1
  Rollers/LConn1 -- Revolute Joint/RConn1
  Rollers/RConn1 -- UP/RConn1
  C/RConn1 -- Transform C to R Ctr/LConn1
  Shaft Conn R/LConn1 -- Link R/RConn2 -- Transform C to R Ctr/RConn1
  "Transform C to R Rear "/RConn1 -- Link R/RConn3
  B/RConn1 -- "Transform C to R Rear "/LConn1

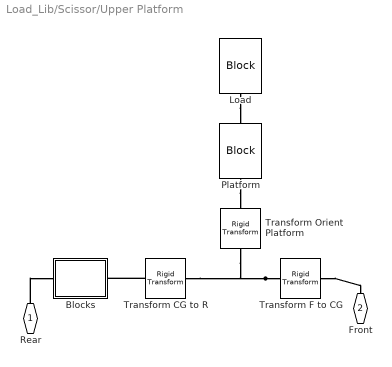
== system Load_Lib/Scissor/Upper Platform ==
  Blocks : Subsystem
  Load : Scissor_Parts_Lib/Block  L=Scissor_Lift_Param.Load.Length  W=Scissor_Lift_Param.Load.Width  H=Scissor_Lift_Param.Load.Height  z_ori=Local +Z  rho=Scissor_Lift_Param.Load.Density  clr=Scissor_Lift_Param.Load.Color  opc=Scissor_Lift_Param.Load.Opacity
  Platform : Scissor_Parts_Lib/Block  L=Scissor_Lift_Param.Upper_Platform.Height  W=Scissor_Lift_Param.Upper_Platform.Width  H=Scissor_Lift_Param.Upper_Platform.Length  z_ori=Local +Z  rho=Scissor_Lift_Param.Upper_Platform.Density  clr=Scissor_Lift_Param.Upper_Platform.Color  opc=Scissor_Lift_Param.Upper_Platform.Opacity
  Transform CG to R : sm_lib/Frames and Transforms/Rigid Transform  RotationMethod=StandardAxis  FollAlignAxisA=+X  BaseAlignAxisA=+Y  FollAlignAxisB=+Y  BaseAlignAxisB=+Z  RotationStandardAxis=+Y  RotationAngle=-90  RotationAngleUnits=deg  RotationArbitraryAxis=[0 0 1]  RotationSequenceAxes=FollowerAxes  RotationSequence=XYX  RotationSequenceAngles=[0 0 0]  RotationSequenceAnglesUnits=deg  RotationMatrix=[1 0 0; 0 1 0; 0 0 1]  Quaternion=[1 0 0 0]  TranslationMethod=Cartesian  TranslationCartesianOffset=[0 0 Scissor_Lift_Param.Link.Length/2]  TranslationCartesianOffsetUnits=cm  TranslationStandardAxis=+Y  TranslationStandardOffset=0  TranslationStandardOffsetUnits=cm  TranslationROffset=0  TranslationROffsetUnits=m  TranslationThetaOffset=0  TranslationThetaOffsetUnits=deg  TranslationZOffset=0  TranslationZOffsetUnits=m
  Transform F to CG : sm_lib/Frames and Transforms/Rigid Transform  RotationMethod=None  FollAlignAxisA=+X  BaseAlignAxisA=+Y  FollAlignAxisB=+Y  BaseAlignAxisB=+Z  RotationStandardAxis=+Z  RotationAngle=0  RotationAngleUnits=deg  RotationArbitraryAxis=[0 0 1]  RotationSequenceAxes=FollowerAxes  RotationSequence=XYX  RotationSequenceAngles=[0 0 0]  RotationSequenceAnglesUnits=deg  RotationMatrix=[1 0 0; 0 1 0; 0 0 1]  Quaternion=[1 0 0 0]  TranslationMethod=Cartesian  TranslationCartesianOffset=[0 0 Scissor_Lift_Param.Link.Length/2]  TranslationCartesianOffsetUnits=cm  TranslationStandardAxis=+Y  TranslationStandardOffset=0  TranslationStandardOffsetUnits=cm  TranslationROffset=0  TranslationROffsetUnits=m  TranslationThetaOffset=0  TranslationThetaOffsetUnits=deg  TranslationZOffset=0  TranslationZOffsetUnits=m
  Transform Orient Platform : sm_lib/Frames and Transforms/Rigid Transform  RotationMethod=StandardAxis  FollAlignAxisA=+X  BaseAlignAxisA=+Y  FollAlignAxisB=+Y  BaseAlignAxisB=+Z  RotationStandardAxis=-X  RotationAngle=90  RotationAngleUnits=deg  RotationArbitraryAxis=[0 0 1]  RotationSequenceAxes=FollowerAxes  RotationSequence=XYX  RotationSequenceAngles=[0 0 0]  RotationSequenceAnglesUnits=deg  RotationMatrix=[1 0 0; 0 1 0; 0 0 1]  Quaternion=[1 0 0 0]  TranslationMethod=None  TranslationCartesianOffset=[0 0 0]  TranslationCartesianOffsetUnits=cm  TranslationStandardAxis=+Y  TranslationStandardOffset=0  TranslationStandardOffsetUnits=cm  TranslationROffset=0  TranslationROffsetUnits=m  TranslationThetaOffset=0  TranslationThetaOffsetUnits=deg  TranslationZOffset=0  TranslationZOffsetUnits=m
  Rear : PMIOPort  Side=Left
  Front : PMIOPort  Port=2  Side=Left
  connections:
  Rear/RConn1 -- Blocks/LConn1
  Transform CG to R/RConn1 -- Blocks/RConn1
  Transform F to CG/LConn1 -- Front/RConn1
  Transform F to CG/RConn1 -- Transform Orient Platform/LConn1 -- Transform CG to R/LConn1
  Platform/LConn1 -- Transform Orient Platform/RConn1
  Load/LConn1 -- Platform/RConn1

== system Load_Lib/Scissor/Actuator/Translational Simscape Intf ==
  Ideal Force Sensor : fl_lib/Mechanical/Mechanical Sensors/Ideal Force Sensor
  Ideal Translational Velocity Source : fl_lib/Mechanical/Mechanical Sources/Ideal Translational Velocity Source
  V : PMIOPort  Side=Right
  F : PMIOPort  Port=2  Side=Left
  R : PMIOPort  Port=3  Side=Right
  C : PMIOPort  Port=4  Side=Left
  connections:
  Ideal Force Sensor/LConn1 -- C/RConn1
  Ideal Translational Velocity Source/RConn2 -- R/RConn1
  Ideal Translational Velocity Source/LConn1 -- Ideal Force Sensor/RConn1
  F/RConn1 -- Ideal Force Sensor/RConn2
  Ideal Translational Velocity Source/RConn1 -- V/RConn1

== system Load_Lib/Scissor/Base/Platform ==
  Block R : Scissor_Parts_Lib/Block  L=Scissor_Lift_Param.Upper_Platform.Length  W=Scissor_Lift_Param.Upper_Platform.Width  H=Scissor_Lift_Param.Upper_Platform.Height  z_ori=Local +Z  rho=Scissor_Lift_Param.Upper_Platform.Density  clr=Scissor_Lift_Param.Upper_Platform.Color  opc=Scissor_Lift_Param.Upper_Platform.Opacity
  Transform Orientation : sm_lib/Frames and Transforms/Rigid Transform  RotationMethod=StandardAxis  FollAlignAxisA=+X  BaseAlignAxisA=+Y  FollAlignAxisB=+Y  BaseAlignAxisB=+Z  RotationStandardAxis=+X  RotationAngle=90  RotationAngleUnits=deg  RotationArbitraryAxis=[0 0 1]  RotationSequenceAxes=FollowerAxes  RotationSequence=XYX  RotationSequenceAngles=[0 0 0]  RotationSequenceAnglesUnits=deg  RotationMatrix=[1 0 0; 0 1 0; 0 0 1]  Quaternion=[1 0 0 0]  TranslationMethod=None  TranslationCartesianOffset=[0 0 0]  TranslationCartesianOffsetUnits=m  TranslationStandardAxis=+X  TranslationStandardOffset=0  TranslationStandardOffsetUnits=m  TranslationROffset=0  TranslationROffsetUnits=m  TranslationThetaOffset=0  TranslationThetaOffsetUnits=deg  TranslationZOffset=0  TranslationZOffsetUnits=m
  Transform Platform CG : sm_lib/Frames and Transforms/Rigid Transform  RotationMethod=StandardAxis  FollAlignAxisA=+X  BaseAlignAxisA=+Y  FollAlignAxisB=+Y  BaseAlignAxisB=+Z  RotationStandardAxis=+Y  RotationAngle=90  RotationAngleUnits=deg  RotationArbitraryAxis=[0 0 1]  RotationSequenceAxes=FollowerAxes  RotationSequence=XYX  RotationSequenceAngles=[0 0 0]  RotationSequenceAnglesUnits=deg  RotationMatrix=[1 0 0; 0 1 0; 0 0 1]  Quaternion=[1 0 0 0]  TranslationMethod=StandardAxis  TranslationCartesianOffset=[0 0 0]  TranslationCartesianOffsetUnits=cm  TranslationStandardAxis=-X  TranslationStandardOffset=Scissor_Lift_Param.Link.Length  TranslationStandardOffsetUnits=cm  TranslationROffset=0  TranslationROffsetUnits=m  TranslationThetaOffset=0  TranslationThetaOffsetUnits=deg  TranslationZOffset=0  TranslationZOffsetUnits=m
  Transform Platform CP : sm_lib/Frames and Transforms/Rigid Transform  RotationMethod=None  FollAlignAxisA=+X  BaseAlignAxisA=+Y  FollAlignAxisB=+Y  BaseAlignAxisB=+Z  RotationStandardAxis=+Y  RotationAngle=0  RotationAngleUnits=deg  RotationArbitraryAxis=[0 0 1]  RotationSequenceAxes=FollowerAxes  RotationSequence=XYX  RotationSequenceAngles=[0 0 0]  RotationSequenceAnglesUnits=deg  RotationMatrix=[1 0 0; 0 1 0; 0 0 1]  Quaternion=[1 0 0 0]  TranslationMethod=Cartesian  TranslationCartesianOffset=[0 -Scissor_Lift_Param.Upper_Platform.Height/2 0]  TranslationCartesianOffsetUnits=cm  TranslationStandardAxis=-Y  TranslationStandardOffset=Scissor_Lift_Param.Roller.Roller_Radius  TranslationStandardOffsetUnits=cm  TranslationROffset=0  TranslationROffsetUnits=m  TranslationThetaOffset=0  TranslationThetaOffsetUnits=deg  TranslationZOffset=0  TranslationZOffsetUnits=m
  S : PMIOPort  Side=Right
  W : PMIOPort  Port=2  Side=Left
  connections:
  Transform Platform CP/LConn1 -- S/RConn1
  Transform Orientation/LConn1 -- W/RConn1
  Transform Platform CG/LConn1 -- Transform Orientation/RConn1 -- Transform Platform CP/RConn1
  Block R/LConn1 -- Transform Platform CG/RConn1

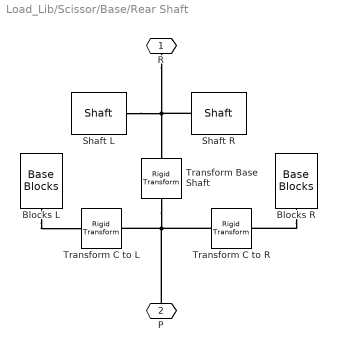
== system Load_Lib/Scissor/Base/Rear Shaft ==
  Blocks L : Scissor_Parts_Lib/Base Blocks  block_length=Scissor_Lift_Param.Base_Block.Length  block_width=Scissor_Lift_Param.Base_Block.Width  block_height=Scissor_Lift_Param.Base_Block.Height  shaft_radius=Scissor_Lift_Param.Roller.Shaft_Radius  shaft_length=Scissor_Lift_Param.Roller.Shaft_Length  material_density=Scissor_Lift_Param.Base_Block.Density  material_color=Scissor_Lift_Param.Base_Block.Color  material_opacity=Scissor_Lift_Param.Base_Block.Opacity
  Blocks R : Scissor_Parts_Lib/Base Blocks  block_length=Scissor_Lift_Param.Base_Block.Length  block_width=Scissor_Lift_Param.Base_Block.Width  block_height=Scissor_Lift_Param.Base_Block.Height  shaft_radius=Scissor_Lift_Param.Roller.Shaft_Radius  shaft_length=Scissor_Lift_Param.Roller.Shaft_Length  material_density=Scissor_Lift_Param.Base_Block.Density  material_color=Scissor_Lift_Param.Base_Block.Color  material_opacity=Scissor_Lift_Param.Base_Block.Opacity
  Shaft L : Scissor_Parts_Lib/Shaft  L=Scissor_Lift_Param.Base_Act_Shaft.Length/2  r=Scissor_Lift_Param.Base_Act_Shaft.Radius  theta=0  z_ori=Local +Z  Ro=Scissor_Lift_Param.Base_Act_Shaft.Density  clr=Scissor_Lift_Param.Base_Act_Shaft.Color  opc=Scissor_Lift_Param.Base_Act_Shaft.Opacity
  Shaft R : Scissor_Parts_Lib/Shaft  L=Scissor_Lift_Param.Base_Act_Shaft.Length/2  r=Scissor_Lift_Param.Base_Act_Shaft.Radius  theta=0  z_ori=Local +Z  Ro=Scissor_Lift_Param.Base_Act_Shaft.Density  clr=Scissor_Lift_Param.Base_Act_Shaft.Color  opc=Scissor_Lift_Param.Base_Act_Shaft.Opacity
  Transform Base Shaft : sm_lib/Frames and Transforms/Rigid Transform  RotationMethod=None  FollAlignAxisA=+X  BaseAlignAxisA=+Y  FollAlignAxisB=+Y  BaseAlignAxisB=+Z  RotationStandardAxis=+Y  RotationAngle=0  RotationAngleUnits=deg  RotationArbitraryAxis=[0 0 1]  RotationSequenceAxes=FollowerAxes  RotationSequence=XYX  RotationSequenceAngles=[0 0 0]  RotationSequenceAnglesUnits=deg  RotationMatrix=[1 0 0; 0 1 0; 0 0 1]  Quaternion=[1 0 0 0]  TranslationMethod=Cartesian  TranslationCartesianOffset=[0 -Scissor_Lift_Param.Base_Block.Height/2 0]  TranslationCartesianOffsetUnits=cm  TranslationStandardAxis=-Y  TranslationStandardOffset=Scissor_Lift_Param.Roller.Roller_Radius  TranslationStandardOffsetUnits=cm  TranslationROffset=0  TranslationROffsetUnits=m  TranslationThetaOffset=0  TranslationThetaOffsetUnits=deg  TranslationZOffset=0  TranslationZOffsetUnits=m
  Transform C to L : sm_lib/Frames and Transforms/Rigid Transform  RotationMethod=None  FollAlignAxisA=+X  BaseAlignAxisA=+Y  FollAlignAxisB=+Y  BaseAlignAxisB=+Z  RotationStandardAxis=+X  RotationAngle=90  RotationAngleUnits=deg  RotationArbitraryAxis=[0 0 1]  RotationSequenceAxes=FollowerAxes  RotationSequence=XYX  RotationSequenceAngles=[0 0 0]  RotationSequenceAnglesUnits=deg  RotationMatrix=[1 0 0; 0 1 0; 0 0 1]  Quaternion=[1 0 0 0]  TranslationMethod=StandardAxis  TranslationCartesianOffset=[0 0 0]  TranslationCartesianOffsetUnits=cm  TranslationStandardAxis=+Z  TranslationStandardOffset=Scissor_Lift_Param.Link_Separation.Outer_Outer/2  TranslationStandardOffsetUnits=cm  TranslationROffset=0  TranslationROffsetUnits=m  TranslationThetaOffset=0  TranslationThetaOffsetUnits=deg  TranslationZOffset=0  TranslationZOffsetUnits=m
  Transform C to R : sm_lib/Frames and Transforms/Rigid Transform  RotationMethod=None  FollAlignAxisA=+X  BaseAlignAxisA=+Y  FollAlignAxisB=+Y  BaseAlignAxisB=+Z  RotationStandardAxis=+X  RotationAngle=90  RotationAngleUnits=deg  RotationArbitraryAxis=[0 0 1]  RotationSequenceAxes=FollowerAxes  RotationSequence=XYX  RotationSequenceAngles=[0 0 0]  RotationSequenceAnglesUnits=deg  RotationMatrix=[1 0 0; 0 1 0; 0 0 1]  Quaternion=[1 0 0 0]  TranslationMethod=StandardAxis  TranslationCartesianOffset=[0 0 0]  TranslationCartesianOffsetUnits=cm  TranslationStandardAxis=-Z  TranslationStandardOffset=Scissor_Lift_Param.Link_Separation.Outer_Outer/2  TranslationStandardOffsetUnits=cm  TranslationROffset=0  TranslationROffsetUnits=m  TranslationThetaOffset=0  TranslationThetaOffsetUnits=deg  TranslationZOffset=0  TranslationZOffsetUnits=m
  R : PMIOPort  Side=Right
  P : PMIOPort  Port=2  Side=Left
  connections:
  Blocks R/LConn1 -- Transform C to R/RConn1
  R/RConn1 -- Shaft L/LConn1 -- Transform Base Shaft/LConn1 -- Shaft R/RConn1
  Blocks L/LConn1 -- Transform C to L/RConn1
  P/RConn1 -- Transform C to L/LConn1 -- Transform Base Shaft/RConn1 -- Transform C to R/LConn1

== system Load_Lib/Scissor/Inner Links/Link Connect ==
  Transform Outer FC : sm_lib/Frames and Transforms/Rigid Transform  RotationMethod=None  FollAlignAxisA=+X  BaseAlignAxisA=+Y  FollAlignAxisB=+Y  BaseAlignAxisB=+Z  RotationStandardAxis=+Z  RotationAngle=0  RotationAngleUnits=deg  RotationArbitraryAxis=[0 0 1]  RotationSequenceAxes=FollowerAxes  RotationSequence=XYX  RotationSequenceAngles=[0 0 0]  RotationSequenceAnglesUnits=deg  RotationMatrix=[1 0 0; 0 1 0; 0 0 1]  Quaternion=[1 0 0 0]  TranslationMethod=StandardAxis  TranslationCartesianOffset=[0 0 0]  TranslationCartesianOffsetUnits=cm  TranslationStandardAxis=+Z  TranslationStandardOffset=Scissor_Lift_Param.Link_Separation.Inner_Inner/2  TranslationStandardOffsetUnits=cm  TranslationROffset=0  TranslationROffsetUnits=m  TranslationThetaOffset=0  TranslationThetaOffsetUnits=deg  TranslationZOffset=0  TranslationZOffsetUnits=m
  Transform Outer FL : sm_lib/Frames and Transforms/Rigid Transform  RotationMethod=None  FollAlignAxisA=+X  BaseAlignAxisA=+Y  FollAlignAxisB=+Y  BaseAlignAxisB=+Z  RotationStandardAxis=+Z  RotationAngle=0  RotationAngleUnits=deg  RotationArbitraryAxis=[0 0 1]  RotationSequenceAxes=FollowerAxes  RotationSequence=XYX  RotationSequenceAngles=[0 0 0]  RotationSequenceAnglesUnits=deg  RotationMatrix=[1 0 0; 0 1 0; 0 0 1]  Quaternion=[1 0 0 0]  TranslationMethod=StandardAxis  TranslationCartesianOffset=[0 0 0]  TranslationCartesianOffsetUnits=cm  TranslationStandardAxis=+Z  TranslationStandardOffset=Scissor_Lift_Param.Link_Separation.Inner_Inner/2  TranslationStandardOffsetUnits=cm  TranslationROffset=0  TranslationROffsetUnits=m  TranslationThetaOffset=0  TranslationThetaOffsetUnits=deg  TranslationZOffset=0  TranslationZOffsetUnits=m
  L : PMIOPort  Side=Right
  C : PMIOPort  Port=2  Side=Left
  R : PMIOPort  Port=3  Side=Right
  connections:
  Transform Outer FL/RConn1 -- L/RConn1
  Transform Outer FC/LConn1 -- R/RConn1
  Transform Outer FC/RConn1 -- C/RConn1 -- Transform Outer FL/LConn1

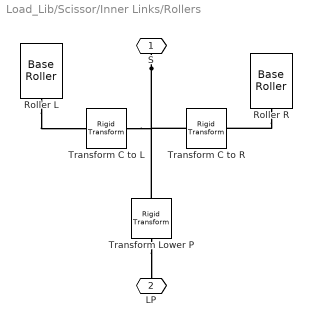
== system Load_Lib/Scissor/Inner Links/Rollers ==
  Roller L : Scissor_Parts_Lib/Base Roller  roller_length=Scissor_Lift_Param.Roller.Roller_Length  roller_radius=Scissor_Lift_Param.Roller.Roller_Radius  shaft_length=Scissor_Lift_Param.Roller.Shaft_Length  shaft_radius=Scissor_Lift_Param.Roller.Shaft_Radius  material_density=Scissor_Lift_Param.Roller.Density  material_color=Scissor_Lift_Param.Roller.Color  material_opacity=Scissor_Lift_Param.Roller.Opacity
  Roller R : Scissor_Parts_Lib/Base Roller  roller_length=Scissor_Lift_Param.Roller.Roller_Length  roller_radius=Scissor_Lift_Param.Roller.Roller_Radius  shaft_length=Scissor_Lift_Param.Roller.Shaft_Length  shaft_radius=Scissor_Lift_Param.Roller.Shaft_Radius  material_density=Scissor_Lift_Param.Roller.Density  material_color=Scissor_Lift_Param.Roller.Color  material_opacity=Scissor_Lift_Param.Roller.Opacity
  Transform C to L : sm_lib/Frames and Transforms/Rigid Transform  RotationMethod=None  FollAlignAxisA=+X  BaseAlignAxisA=+Y  FollAlignAxisB=+Y  BaseAlignAxisB=+Z  RotationStandardAxis=+X  RotationAngle=90  RotationAngleUnits=deg  RotationArbitraryAxis=[0 0 1]  RotationSequenceAxes=FollowerAxes  RotationSequence=XYX  RotationSequenceAngles=[0 0 0]  RotationSequenceAnglesUnits=deg  RotationMatrix=[1 0 0; 0 1 0; 0 0 1]  Quaternion=[1 0 0 0]  TranslationMethod=StandardAxis  TranslationCartesianOffset=[0 0 0]  TranslationCartesianOffsetUnits=cm  TranslationStandardAxis=+Z  TranslationStandardOffset=Scissor_Lift_Param.Link_Separation.Inner_Inner/2  TranslationStandardOffsetUnits=cm  TranslationROffset=0  TranslationROffsetUnits=m  TranslationThetaOffset=0  TranslationThetaOffsetUnits=deg  TranslationZOffset=0  TranslationZOffsetUnits=m
  Transform C to R : sm_lib/Frames and Transforms/Rigid Transform  RotationMethod=None  FollAlignAxisA=+X  BaseAlignAxisA=+Y  FollAlignAxisB=+Y  BaseAlignAxisB=+Z  RotationStandardAxis=+X  RotationAngle=90  RotationAngleUnits=deg  RotationArbitraryAxis=[0 0 1]  RotationSequenceAxes=FollowerAxes  RotationSequence=XYX  RotationSequenceAngles=[0 0 0]  RotationSequenceAnglesUnits=deg  RotationMatrix=[1 0 0; 0 1 0; 0 0 1]  Quaternion=[1 0 0 0]  TranslationMethod=StandardAxis  TranslationCartesianOffset=[0 0 0]  TranslationCartesianOffsetUnits=cm  TranslationStandardAxis=-Z  TranslationStandardOffset=Scissor_Lift_Param.Link_Separation.Inner_Inner/2  TranslationStandardOffsetUnits=cm  TranslationROffset=0  TranslationROffsetUnits=m  TranslationThetaOffset=0  TranslationThetaOffsetUnits=deg  TranslationZOffset=0  TranslationZOffsetUnits=m
  Transform Lower P : sm_lib/Frames and Transforms/Rigid Transform  RotationMethod=StandardAxis  FollAlignAxisA=+X  BaseAlignAxisA=+Y  FollAlignAxisB=+Y  BaseAlignAxisB=+Z  RotationStandardAxis=+Y  RotationAngle=-90  RotationAngleUnits=deg  RotationArbitraryAxis=[0 0 1]  RotationSequenceAxes=FollowerAxes  RotationSequence=XYX  RotationSequenceAngles=[0 0 0]  RotationSequenceAnglesUnits=deg  RotationMatrix=[1 0 0; 0 1 0; 0 0 1]  Quaternion=[1 0 0 0]  TranslationMethod=Cartesian  TranslationCartesianOffset=[0 Scissor_Lift_Param.Base_Block.Height/2 0]  TranslationCartesianOffsetUnits=cm  TranslationStandardAxis=-Y  TranslationStandardOffset=Scissor_Lift_Param.Roller.Roller_Radius  TranslationStandardOffsetUnits=cm  TranslationROffset=0  TranslationROffsetUnits=m  TranslationThetaOffset=0  TranslationThetaOffsetUnits=deg  TranslationZOffset=0  TranslationZOffsetUnits=m
  S : PMIOPort  Side=Right
  LP : PMIOPort  Port=2  Side=Left
  connections:
  Transform Lower P/LConn1 -- LP/RConn1
  Roller R/RConn1 -- Transform C to R/RConn1
  S/RConn1 -- Transform Lower P/RConn1 -- Transform C to R/LConn1 -- Transform C to L/LConn1
  Roller L/RConn1 -- Transform C to L/RConn1

== system Load_Lib/Scissor/Inner Links/Shaft Actuator ==
  Shaft L : Scissor_Parts_Lib/Shaft  L=Scissor_Lift_Param.Link_Act_Shaft.Length/2  r=Scissor_Lift_Param.Link_Act_Shaft.Radius  theta=0  z_ori=Local +Z  Ro=Scissor_Lift_Param.Link_Act_Shaft.Density  clr=Scissor_Lift_Param.Colors.Yellow  opc=Scissor_Lift_Param.Link_Act_Shaft.Opacity
  Shaft R : Scissor_Parts_Lib/Shaft  L=Scissor_Lift_Param.Link_Act_Shaft.Length/2  r=Scissor_Lift_Param.Link_Act_Shaft.Radius  theta=0  z_ori=Local +Z  Ro=Scissor_Lift_Param.Link_Act_Shaft.Density  clr=Scissor_Lift_Param.Colors.Yellow  opc=Scissor_Lift_Param.Link_Act_Shaft.Opacity
  Transform Act Shaft : sm_lib/Frames and Transforms/Rigid Transform  RotationMethod=None  FollAlignAxisA=+X  BaseAlignAxisA=+Y  FollAlignAxisB=+Y  BaseAlignAxisB=+Z  RotationStandardAxis=+X  RotationAngle=90  RotationAngleUnits=deg  RotationArbitraryAxis=[0 0 1]  RotationSequenceAxes=FollowerAxes  RotationSequence=XYX  RotationSequenceAngles=[0 0 0]  RotationSequenceAnglesUnits=deg  RotationMatrix=[1 0 0; 0 1 0; 0 0 1]  Quaternion=[1 0 0 0]  TranslationMethod=StandardAxis  TranslationCartesianOffset=[0 0 0]  TranslationCartesianOffsetUnits=cm  TranslationStandardAxis=-X  TranslationStandardOffset=Scissor_Lift_Param.Link_Act_Shaft.Offset  TranslationStandardOffsetUnits=cm  TranslationROffset=0  TranslationROffsetUnits=m  TranslationThetaOffset=0  TranslationThetaOffsetUnits=deg  TranslationZOffset=0  TranslationZOffsetUnits=m
  Act : PMIOPort  Side=Right
  UP : PMIOPort  Port=2  Side=Left
  connections:
  Transform Act Shaft/LConn1 -- UP/RConn1
  Act/RConn1 -- Transform Act Shaft/RConn1 -- Shaft L/LConn1 -- Shaft R/RConn1
